simulink model "PId_deploy_hw"  (R2025a)
settings: Solver=ode4  StartTime=0.0  StopTime=inf  FixedStep=Ts  RelTol=1e-3  EnableMultiTasking=on
InitFcn:
  | addpath('functions');
model workspace (MATLAB code in the model file):
  | arm_torque = 0;
  | L_arm = 0.2;
  | I_arm = 0.01;
  | lcom_1 = 0.6;
  | I_1 = 0.02;
  | m_1 = 1;
  | L_1 = 1;
  | 
  | init_cond = [pi/2; 0; 0.01; 0];
undefined symbols (not defined in the file or in its folder): DiscIntNeverNeededParam, Ts
settings Model: Creator=Esther  LastModifiedBy=marcus
settings OptimizationCC: DefaultParameterBehavior=Inlined  EnhancedBackFolding=on  PassReuseOutputArgsAs=Individual arguments  ZeroExternalMemoryAtStartup=off  ZeroInternalMemoryAtStartup=off  MaxStackSize=64  OptimizeBlockOrder=speed  DifferentSizesBufferReuse=on  OptimizationCustomize=off  EfficientTunableParamExpr=on
settings DebuggingCC: ParameterTunabilityLossMsg=error
settings HardwareCC: ProdBitPerPointer=32.0  ProdBitPerSizeT=32.0  ProdBitPerPtrDiffT=32.0  ProdLargestAtomicInteger=Long  ProdLargestAtomicFloat=Double  ProdWordSize=32.0  ProdLongLongMode=on  ProdHWDeviceType=ARM Compatible->ARM Cortex-M
settings RTWCC: SystemTargetFile=ert.tlc  TemplateMakefile=ert_default_tmf  Toolchain=Armclang Compiler  Description=Embedded Coder
settings CodeAppCC: ForceParamTrailComments=on  IgnoreCustomStorageClasses=off  OperatorAnnotations=on  SimulinkDataObjDesc=on  SFDataObjDesc=on  InsertBlockDesc=on
settings ERTTargetCC: ExtModeTransport=3.0  ExtModeStaticAllocSize=2048.0  ERTCustomFileTemplate=example_file_process.tlc  TargetLangStandard=C99 (ISO)  CodeReplacementLibrary=ARM Cortex-M

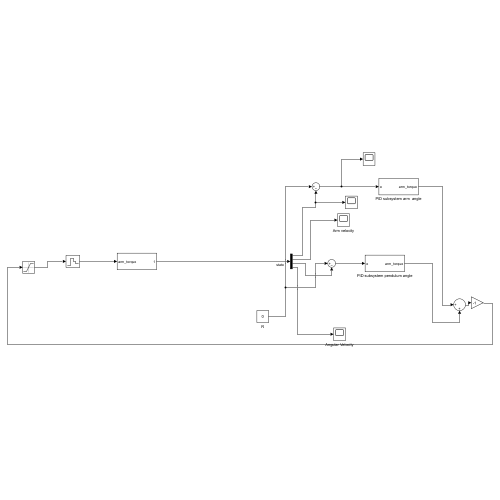
[thumbnail: Simulink's stored preview of the top-level diagram]
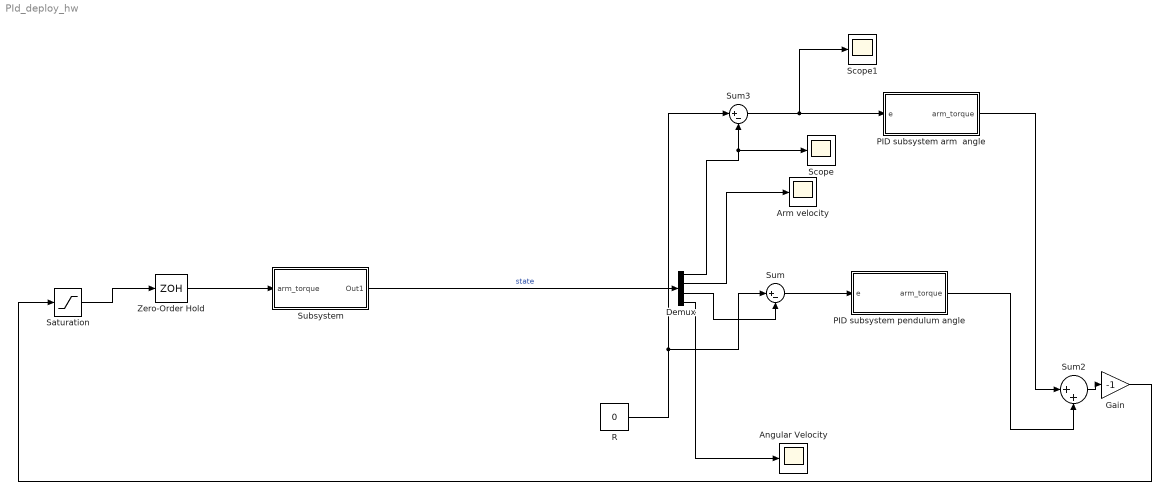
== system PId_deploy_hw ==
  Angular Velocity : Scope
      settings: ActiveDisplayYMinimum=-3875.8658390527003  ActiveDisplayYMaximum=3642.7464695660938  DataLoggingVariableName=ScopeData2
  Arm velocity : Scope
      settings: DataLoggingVariableName=ScopeData4
  Demux : Demux
  Gain : Gain  Gain=-1
  PID subsystem arm  angle : Subsystem
  PID subsystem pendulum angle : Subsystem
  R : Constant  Value=0
  Saturation : Saturate
  Scope : Scope
      settings: ActiveDisplayYMinimum=-0.209246368939112  ActiveDisplayYMaximum=0.21172316816115397
  Scope1 : Scope
      settings: ActiveDisplayYMinimum=-2.0998482153915092  ActiveDisplayYMaximum=0.23939956718142349  DataLoggingVariableName=ScopeData3
  Subsystem : Subsystem
  Sum : Sum  Inputs=|+-
  Sum2 : Sum  Inputs=|++
  Sum3 : Sum  Inputs=|+-
  Zero-Order Hold : ZeroOrderHold  SampleTime=Ts
  wires:
  Subsystem/1(Out1) -> Demux/1  "state"
  R/1 -> Sum/1, Sum3/1
  Demux/3 -> Sum/2
  Demux/4 -> Angular Velocity/1
  Sum2/1 -> Gain/1
  PID subsystem arm  angle/1(arm_torque) -> Sum2/1
  Demux/1 -> Scope/1, Sum3/2
  Demux/2 -> Arm velocity/1
  Zero-Order Hold/1 -> Subsystem/1(arm_torque)
  Sum/1 -> PID subsystem pendulum angle/1(e)
  Sum3/1 -> Scope1/1, PID subsystem arm  angle/1(e)
  Gain/1 -> Saturation/1
  PID subsystem pendulum angle/1(arm_torque) -> Sum2/2
  Saturation/1 -> Zero-Order Hold/1

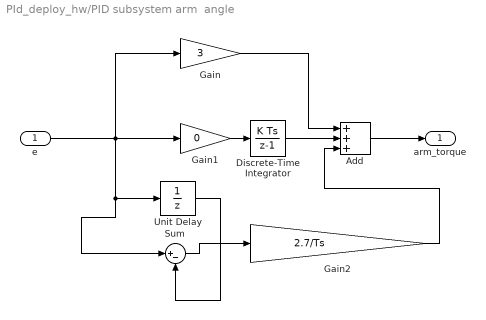
== system PId_deploy_hw/PID subsystem arm  angle ==
  e : Inport
  Add : Sum  Inputs=+++
  Discrete-Time Integrator : DiscreteIntegrator  gainval=1  SampleTime=Ts  ICPrevOutput=DiscIntNeverNeededParam  ICPrevScaledInput=DiscIntNeverNeededParam
  Gain : Gain  Gain=3
  Gain1 : Gain  Gain=0
  Gain2 : Gain  Gain=2.7/Ts
  Sum : Sum  Inputs=|+-
  Unit Delay : UnitDelay  SampleTime=-1  HasFrameUpgradeWarning=on
  arm_torque : Outport
  wires:
  e/1 -> Sum/1, Unit Delay/1, Gain/1, Gain1/1
  Unit Delay/1 -> Sum/2
  Discrete-Time Integrator/1 -> Add/2
  Gain/1 -> Add/1
  Add/1 -> arm_torque/1
  Gain1/1 -> Discrete-Time Integrator/1
  Gain2/1 -> Add/3
  Sum/1 -> Gain2/1

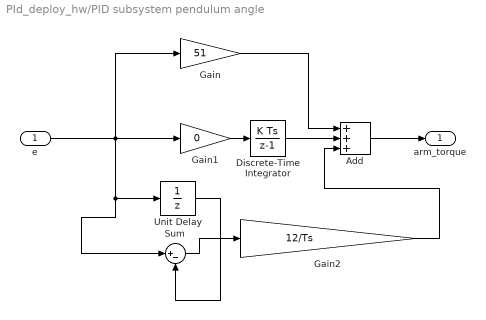
== system PId_deploy_hw/PID subsystem pendulum angle ==
  e : Inport
  Add : Sum  Inputs=+++
  Discrete-Time Integrator : DiscreteIntegrator  gainval=1  SampleTime=Ts  ICPrevOutput=DiscIntNeverNeededParam  ICPrevScaledInput=DiscIntNeverNeededParam
  Gain : Gain  Gain=51
  Gain1 : Gain  Gain=0
  Gain2 : Gain  Gain=12/Ts
  Sum : Sum  Inputs=|+-
  Unit Delay : UnitDelay  SampleTime=-1  HasFrameUpgradeWarning=on
  arm_torque : Outport
  wires:
  e/1 -> Sum/1, Unit Delay/1, Gain/1, Gain1/1
  Unit Delay/1 -> Sum/2
  Discrete-Time Integrator/1 -> Add/2
  Gain/1 -> Add/1
  Add/1 -> arm_torque/1
  Gain1/1 -> Discrete-Time Integrator/1
  Gain2/1 -> Add/3
  Sum/1 -> Gain2/1

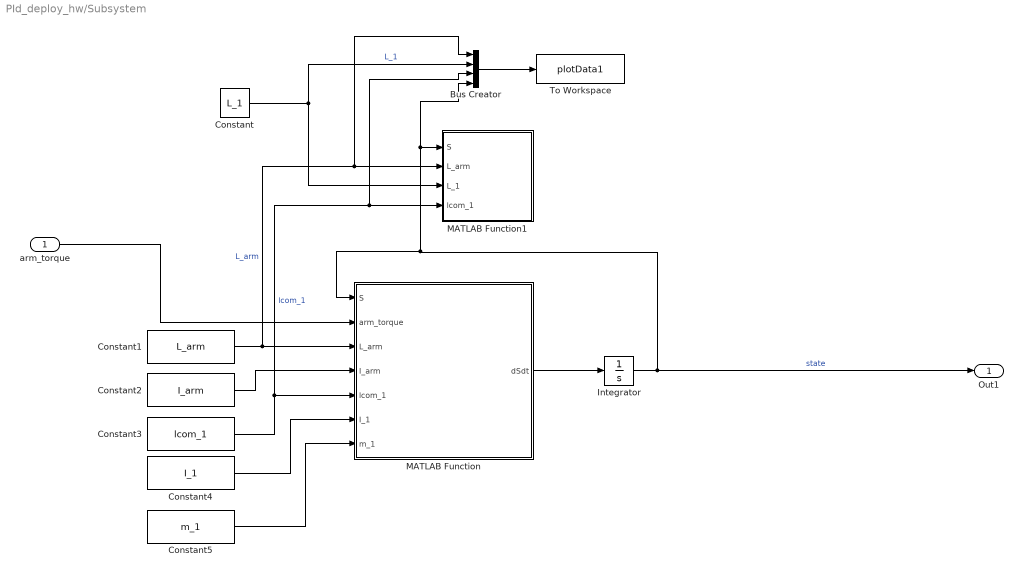
== system PId_deploy_hw/Subsystem ==
  arm_torque : Inport
  Bus Creator : BusCreator  Inputs=4
  Constant : Constant  Value=L_1
  Constant1 : Constant  Value=L_arm
  Constant2 : Constant  Value=I_arm
  Constant3 : Constant  Value=lcom_1
  Constant4 : Constant  Value=I_1
  Constant5 : Constant  Value=m_1
  Integrator : Integrator  InitialCondition=init_cond
  MATLAB Function : MATLAB Function  TreatAsAtomicUnit=on
  MATLAB Function1 : MATLAB Function  TreatAsAtomicUnit=on
  To Workspace : ToWorkspace  VariableName=plotData1  SaveFormat=Timeseries  SampleTime=-1
  Out1 : Outport
  wires:
  Bus Creator/1 -> To Workspace/1
  Constant/1 -> Bus Creator/2, MATLAB Function1/3(L_1)  "L_1"
  Constant2/1 -> MATLAB Function/4(I_arm)
  Constant4/1 -> MATLAB Function/6(I_1)
  Constant1/1 -> MATLAB Function/3(L_arm), Bus Creator/1, MATLAB Function1/2(L_arm)  "L_arm"
  Integrator/1 -> Out1/1, MATLAB Function/1(S), MATLAB Function1/1(S), Bus Creator/4  "state"
  Constant3/1 -> Bus Creator/3, MATLAB Function1/4(lcom_1), MATLAB Function/5(lcom_1)  "lcom_1"
  Constant5/1 -> MATLAB Function/7(m_1)
  arm_torque/1 -> MATLAB Function/2(arm_torque)
  MATLAB Function/1(dSdt) -> Integrator/1

== matlab function PId_deploy_hw/Subsystem/MATLAB Function ==
  data: S input size=4; dSdt output size=4; arm_torque input size=1; L_arm input size=1; I_arm input size=1; lcom_1 input size=1; I_1 input size=1; m_1 input size=1
function dSdt = get_dSdt(S, arm_torque, L_arm, I_arm, lcom_1, I_1, m_1)
    t = 0;
    g = 9.81;
    phys_param = [L_arm, I_arm, lcom_1, I_1, m_1, g];
    fric_arm = [0.018, 0.018, 100];
    fric_1 = [0.0001, 0.0001, 100];
    dSdt = furuta_single_state_derivative(t, S, arm_torque, phys_param, fric_arm, fric_1);
end

== matlab function PId_deploy_hw/Subsystem/MATLAB Function1 ==
  settings: updateMethod=DISCRETE
  data: S input; L_arm input; L_1 input; lcom_1 input
function animation(S, L_arm, L_1, lcom_1)
    update_ratio = 100;
    realtime_animation_single(S, L_arm, L_1, lcom_1, update_ratio);
end
